simulink model "demo_array_faults"  (R2026a)
settings: Solver=FixedStepDiscrete  StopTime=4  FixedStep=1
settings Model: Creator=harry_31916  LastModifiedBy=harry_31916

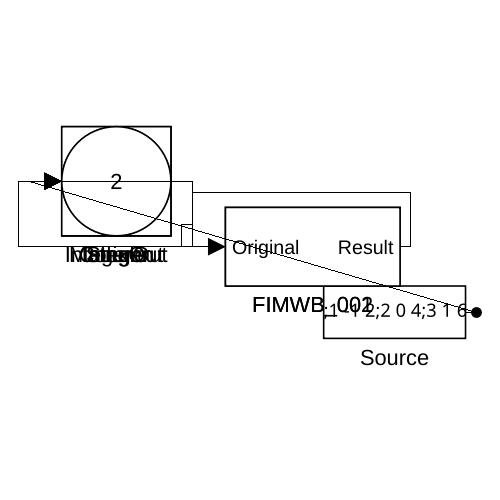
[thumbnail: Simulink's stored preview of the top-level diagram]
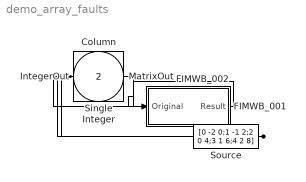
== system demo_array_faults ==
  Column : Reshape  OutputDimensionality=Column vector (2-D)
  FIMWB_001 : Subsystem  Tag=fimwb.fault.1
  FIMWB_002 : Subsystem  Tag=fimwb.fault.2
  Integer : DataTypeConversion  OutDataTypeStr=int64
  Single : DataTypeConversion  OutDataTypeStr=single
  Source : FromWorkspace  VariableName=[0 -2 0;1 -1 2;2 0 4;3 1 6;4 2 8]  SampleTime=1  Interpolate=off  OutputAfterFinalValue=Holding final value
  MatrixOut : Outport
  IntegerOut : Outport  Port=2
  wires:
  Source/1 -> Column/1, Integer/1
  Column/1 -> Single/1
  Single/1 -> FIMWB_001/1(Original)
  FIMWB_001/1(Result) -> MatrixOut/1
  Integer/1 -> FIMWB_002/1(Original)
  FIMWB_002/1(Result) -> IntegerOut/1

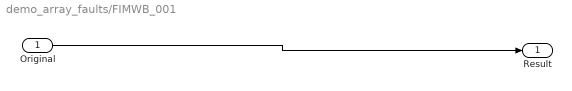
== system demo_array_faults/FIMWB_001 ==
  Original : Inport
  Result : Outport
  wires:
  Original/1 -> Result/1

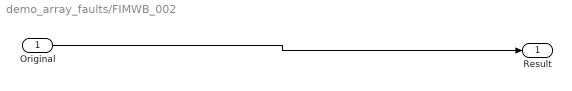
== system demo_array_faults/FIMWB_002 ==
  Original : Inport
  Result : Outport
  wires:
  Original/1 -> Result/1
